simulink library "casper_library_pfbs"  (Simulink 7.2)
settings: Solver=ode45  SolverMode=SingleTasking  StartTime=0.0  StopTime=10.0  RelTol=1e-3
undefined symbols (not defined in the file or in its folder): pfb_coeff_gen_calc
libraries: xbsIndex_r4 x138, casper_library_pfbs x18, casper_library_delays x9, casper_library_misc x7, casper_library_flow_control x2
(part 3 of 3)

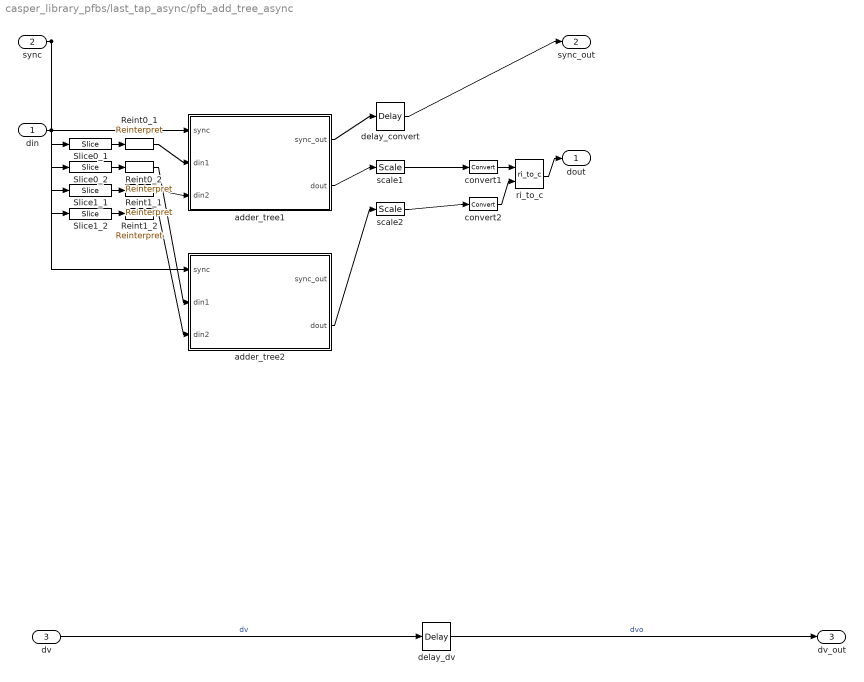
== system casper_library_pfbs/last_tap_async/pfb_add_tree_async ==
  din : Inport
  sync : Inport  Port=2
  dv : Inport  Port=3
  Reint0_1 : xbsIndex_r4/Reinterpret  force_arith_type=on  arith_type="Signed  (2's comp)"  force_bin_pt=on  bin_pt=coeff_bits + data_in_bits - 2  block_type=reinterpret
      settings: infoedit="Changes signal type without altering the binary representation.   You can changed the signal between signed and unsigned, and relocate the binary point.<br><br>Hardware notes: In hardware this block costs nothing.<br><br>Example:  Suppose the input is 6 bits wide, signed, with 2 fractional bits, and the output is forced to unsigned with 0 fractional bits.  Then an input of -2.0 (1110.00 in binary 2's complement) becomes an output of 56 (111000 in binary)."
  Reint0_2 : xbsIndex_r4/Reinterpret  force_arith_type=on  arith_type="Signed  (2's comp)"  force_bin_pt=on  bin_pt=coeff_bits + data_in_bits - 2  block_type=reinterpret
      settings: infoedit="Changes signal type without altering the binary representation.   You can changed the signal between signed and unsigned, and relocate the binary point.<br><br>Hardware notes: In hardware this block costs nothing.<br><br>Example:  Suppose the input is 6 bits wide, signed, with 2 fractional bits, and the output is forced to unsigned with 0 fractional bits.  Then an input of -2.0 (1110.00 in binary 2's complement) becomes an output of 56 (111000 in binary)."
  Reint1_1 : xbsIndex_r4/Reinterpret  force_arith_type=on  arith_type="Signed  (2's comp)"  force_bin_pt=on  bin_pt=coeff_bits + data_in_bits - 2  block_type=reinterpret
      settings: infoedit="Changes signal type without altering the binary representation.   You can changed the signal between signed and unsigned, and relocate the binary point.<br><br>Hardware notes: In hardware this block costs nothing.<br><br>Example:  Suppose the input is 6 bits wide, signed, with 2 fractional bits, and the output is forced to unsigned with 0 fractional bits.  Then an input of -2.0 (1110.00 in binary 2's complement) becomes an output of 56 (111000 in binary)."
  Reint1_2 : xbsIndex_r4/Reinterpret  force_arith_type=on  arith_type="Signed  (2's comp)"  force_bin_pt=on  bin_pt=coeff_bits + data_in_bits - 2  block_type=reinterpret
      settings: infoedit="Changes signal type without altering the binary representation.   You can changed the signal between signed and unsigned, and relocate the binary point.<br><br>Hardware notes: In hardware this block costs nothing.<br><br>Example:  Suppose the input is 6 bits wide, signed, with 2 fractional bits, and the output is forced to unsigned with 0 fractional bits.  Then an input of -2.0 (1110.00 in binary 2's complement) becomes an output of 56 (111000 in binary)."
  Slice0_1 : xbsIndex_r4/Slice  nbits=coeff_bits + data_in_bits  boolean_output=off  mode=Upper Bit Location + Width  bit1=0  base1=MSB of Input  bit0=0  base0=MSB of Input  dbl_ovrd=off  block_type=slice
  Slice0_2 : xbsIndex_r4/Slice  nbits=coeff_bits + data_in_bits  boolean_output=off  mode=Upper Bit Location + Width  bit1=-16  base1=MSB of Input  bit0=0  base0=MSB of Input  dbl_ovrd=off  block_type=slice
  Slice1_1 : xbsIndex_r4/Slice  nbits=coeff_bits + data_in_bits  boolean_output=off  mode=Upper Bit Location + Width  bit1=-32  base1=MSB of Input  bit0=0  base0=MSB of Input  dbl_ovrd=off  block_type=slice
  Slice1_2 : xbsIndex_r4/Slice  nbits=coeff_bits + data_in_bits  boolean_output=off  mode=Upper Bit Location + Width  bit1=-48  base1=MSB of Input  bit0=0  base0=MSB of Input  dbl_ovrd=off  block_type=slice
  adder_tree1 : Subsystem  AncestorBlock=casper_library_misc/adder_tree  mask(adder_tree){n_inputs=2, latency=add_latency, adder_imp=Fabric, first_stage_hdl=off}
      mask prompts: n_inputs "Number of Inputs"; latency "Add Latency"; adder_imp "Adder implementation"; first_stage_hdl "Use behavioural HDL for first stage of adders"
      mask help:
      | Sums all inputs using a tree of adds and delays.
      |
      | Number of inputs: The number of inputs to the block to be summed
      | Add latency: The number of clock cycles to perform one addition (affects timing)..
      | Adder implementation: choice of fabric or DSP48E core, or behavioral HDL
      | Use behavioural HDL for first stage of adders: Causes the first stage of adders to be absorbed into DSP blocks if multipliers precede them (Virtex 5). Overrides Adder implementation
      mask init:
      | adder_tree_init(gcb, ...
      |     'n_inputs', n_inputs, ...
      |     'latency', latency, ...
      |     'adder_imp', adder_imp, ...
      |     'first_stage_hdl', first_stage_hdl);
      settings: AttributesFormatString=latency 1
      mask Help: eval('xlWeb(''http://casper.berkeley.edu/wiki/Adder_tree'')')
      mask StyleString: edit,edit,popup(Behavioral|Fabric|DSP48),checkbox
  adder_tree2 : Subsystem  AncestorBlock=casper_library_misc/adder_tree  mask(adder_tree){n_inputs=2, latency=add_latency, adder_imp=Fabric, first_stage_hdl=off}
      mask prompts: n_inputs "Number of Inputs"; latency "Add Latency"; adder_imp "Adder implementation"; first_stage_hdl "Use behavioural HDL for first stage of adders"
      mask help:
      | Sums all inputs using a tree of adds and delays.
      |
      | Number of inputs: The number of inputs to the block to be summed
      | Add latency: The number of clock cycles to perform one addition (affects timing)..
      | Adder implementation: choice of fabric or DSP48E core, or behavioral HDL
      | Use behavioural HDL for first stage of adders: Causes the first stage of adders to be absorbed into DSP blocks if multipliers precede them (Virtex 5). Overrides Adder implementation
      mask init:
      | adder_tree_init(gcb, ...
      |     'n_inputs', n_inputs, ...
      |     'latency', latency, ...
      |     'adder_imp', adder_imp, ...
      |     'first_stage_hdl', first_stage_hdl);
      settings: AttributesFormatString=latency 1
      mask Help: eval('xlWeb(''http://casper.berkeley.edu/wiki/Adder_tree'')')
      mask StyleString: edit,edit,popup(Behavioral|Fabric|DSP48),checkbox
  convert1 : xbsIndex_r4/Convert  gui_display_data_type=Fixed-point  arith_type="Signed  (2's comp)"  n_bits=data_out_bits  bin_pt=data_out_bits-1  float_type=Single  exp_bits=8  fraction_bits=24  quantization=Truncate  overflow=Saturate  en=off  latency=add_latency  dbl_ovrd=off  pipeline=on  block_type=convert
      settings: block_version=11.4
  convert2 : xbsIndex_r4/Convert  gui_display_data_type=Fixed-point  arith_type="Signed  (2's comp)"  n_bits=data_out_bits  bin_pt=data_out_bits-1  float_type=Single  exp_bits=8  fraction_bits=24  quantization=Truncate  overflow=Saturate  en=off  latency=add_latency  dbl_ovrd=off  pipeline=on  block_type=convert
      settings: block_version=11.4
  delay_convert : xbsIndex_r4/Delay  rst=off  infoeditControl=Selection of Reset will increase slice count due to use of real FFs and instead of SRLs  en=off  latency=add_latency  dbl_ovrd=off  reg_retiming=off  block_type=delay
      settings: block_version=11.4
  delay_dv : xbsIndex_r4/Delay  rst=off  infoeditControl=Selection of Reset will increase slice count due to use of real FFs and instead of SRLs  en=off  latency=2  dbl_ovrd=off  reg_retiming=off  block_type=delay
      settings: block_version=11.4
  ri_to_c : casper_library_misc/ri_to_c
  scale1 : xbsIndex_r4/Scale  scale_factor=-2  dbl_ovrd=off  block_type=scale
  scale2 : xbsIndex_r4/Scale  scale_factor=-2  dbl_ovrd=off  block_type=scale
  dout : Outport
  sync_out : Outport  Port=2
  dv_out : Outport  Port=3
  wires:
  dv/1 -> delay_dv/1  "dv"
  delay_dv/1 -> dv_out/1  "dvo"
  adder_tree1/2(dout) -> scale1/1
  scale1/1 -> convert1/1
  adder_tree2/2(dout) -> scale2/1
  scale2/1 -> convert2/1
  convert1/1 -> ri_to_c/1
  convert2/1 -> ri_to_c/2
  ri_to_c/1 -> dout/1
  sync/1 -> adder_tree1/1(sync), adder_tree2/1(sync)
  adder_tree1/1(sync_out) -> delay_convert/1
  delay_convert/1 -> sync_out/1
  din/1 -> Slice0_1/1, Slice0_2/1, Slice1_1/1, Slice1_2/1
  Slice0_1/1 -> Reint0_1/1
  Reint0_1/1 -> adder_tree1/2(din1)
  Slice0_2/1 -> Reint0_2/1
  Reint0_2/1 -> adder_tree2/2(din1)
  Slice1_1/1 -> Reint1_1/1
  Reint1_1/1 -> adder_tree1/3(din2)
  Slice1_2/1 -> Reint1_2/1
  Reint1_2/1 -> adder_tree2/3(din2)

== system casper_library_pfbs/last_tap_async/ri_to_c ==
  re : Inport
  im : Inport  Port=2
  Concat : xbsIndex_r4/Concat  num_inputs=2  dbl_ovrd=off  block_type=concat
      settings: block_version=9.1.01
  Reinterpret : xbsIndex_r4/Reinterpret  force_arith_type=on  arith_type=Unsigned  force_bin_pt=on  bin_pt=0  block_type=reinterpret
      settings: infoedit="Changes signal type without altering the binary representation.   You can changed the signal between signed and unsigned, and relocate the binary point.<P><P>Hardware notes: In hardware this block costs nothing.<P><P>Example:  Suppose the input is 6 bits wide, signed, with 2 fractional bits, and the output is forced to unsigned with 0 fractional bits.  Then an input of -2.0 (1110.00 in binary 2's complement) becomes an output of 56 (111000 in binary)."  block_version=9.1.01
  Reinterpret1 : xbsIndex_r4/Reinterpret  force_arith_type=on  arith_type=Unsigned  force_bin_pt=on  bin_pt=0  block_type=reinterpret
      settings: infoedit="Changes signal type without altering the binary representation.   You can changed the signal between signed and unsigned, and relocate the binary point.<P><P>Hardware notes: In hardware this block costs nothing.<P><P>Example:  Suppose the input is 6 bits wide, signed, with 2 fractional bits, and the output is forced to unsigned with 0 fractional bits.  Then an input of -2.0 (1110.00 in binary 2's complement) becomes an output of 56 (111000 in binary)."  block_version=9.1.01
  c : Outport
  wires:
  im/1 -> Reinterpret1/1
  Concat/1 -> c/1
  re/1 -> Reinterpret/1
  Reinterpret1/1 -> Concat/2
  Reinterpret/1 -> Concat/1

== system casper_library_pfbs/pfb_fir_async/sync_generate ==
  sync : Inport
  dv : Inport  Port=2
  Constant : xbsIndex_r4/Constant  const=1  gui_display_data_type=Fixed-point  arith_type=Boolean  n_bits=16  bin_pt=14  preci_type=Single  exp_width=8  frac_width=24  explicit_period=on  period=1  equ=P=C  opselect=C  inp2=PCIN>>17  opr=+  inp1=P  carry=CIN  dbl_ovrd=off  block_type=constant
      settings: block_version=11.4
  Constant1 : xbsIndex_r4/Constant  const=(2^(pfb_bits - simul_bits) * (total_taps-1))+1  gui_display_data_type=Fixed-point  arith_type=Unsigned  n_bits=32  bin_pt=0  preci_type=Single  exp_width=8  frac_width=24  explicit_period=off  period=1  equ=P=C  opselect=C  inp2=PCIN>>17  opr=+  inp1=P  carry=CIN  dbl_ovrd=off  block_type=constant
      settings: block_version=11.4
  Counter : xbsIndex_r4/Counter  cnt_type=Free Running  cnt_to=Inf  operation=Up  start_count=0  cnt_by_val=1  arith_type=Unsigned  n_bits=32  bin_pt=0  load_pin=off  rst=on  en=on  explicit_period=on  period=1  dbl_ovrd=off  use_behavioral_HDL=off  implementation=Fabric  block_type=counter
      settings: block_version=11.4
  Logical : xbsIndex_r4/Logical  logical_function=AND  inputs=2  en=off  latency=0  precision=Full  arith_type=Unsigned  n_bits=16  bin_pt=0  align_bp=on  dbl_ovrd=off  block_type=logical
      settings: block_version=11.4
  Register : xbsIndex_r4/Register  init=0  rst=on  en=on  dbl_ovrd=off  block_type=register
      settings: block_version=11.4
  Relational : xbsIndex_r4/Relational  mode=a=b  en=off  latency=1  dbl_ovrd=off  block_type=relational
  sync_delay : xbsIndex_r4/Delay  rst=off  infoeditControl=Selection of Reset will increase slice count due to use of real FFs and instead of SRLs  en=off  latency=(bram_latency * (total_taps-1)) - 3  dbl_ovrd=off  reg_retiming=off  block_type=delay
      settings: block_version=11.4
  sync_out : Outport
  wires:
  sync_delay/1 -> sync_out/1
  dv/1 -> Logical/1
  sync/1 -> Register/3
  Relational/1 -> sync_delay/1, Counter/1, Register/2  "sync_out"
  Constant1/1 -> Relational/2
  Counter/1 -> Relational/1
  Logical/1 -> Counter/2
  Register/1 -> Logical/2
  Constant/1 -> Register/1

== system casper_library_pfbs/tap/ri_to_c ==
  re : Inport
  im : Inport  Port=2
  Concat : xbsIndex_r4/Concat  num_inputs=2  dbl_ovrd=off  block_type=concat
      settings: block_version=9.1.01
  Reinterpret : xbsIndex_r4/Reinterpret  force_arith_type=on  arith_type=Unsigned  force_bin_pt=on  bin_pt=0  block_type=reinterpret
      settings: infoedit="Changes signal type without altering the binary representation.   You can changed the signal between signed and unsigned, and relocate the binary point.<P><P>Hardware notes: In hardware this block costs nothing.<P><P>Example:  Suppose the input is 6 bits wide, signed, with 2 fractional bits, and the output is forced to unsigned with 0 fractional bits.  Then an input of -2.0 (1110.00 in binary 2's complement) becomes an output of 56 (111000 in binary)."  block_version=9.1.01
  Reinterpret1 : xbsIndex_r4/Reinterpret  force_arith_type=on  arith_type=Unsigned  force_bin_pt=on  bin_pt=0  block_type=reinterpret
      settings: infoedit="Changes signal type without altering the binary representation.   You can changed the signal between signed and unsigned, and relocate the binary point.<P><P>Hardware notes: In hardware this block costs nothing.<P><P>Example:  Suppose the input is 6 bits wide, signed, with 2 fractional bits, and the output is forced to unsigned with 0 fractional bits.  Then an input of -2.0 (1110.00 in binary 2's complement) becomes an output of 56 (111000 in binary)."  block_version=9.1.01
  c : Outport
  wires:
  im/1 -> Reinterpret1/1
  Concat/1 -> c/1
  re/1 -> Reinterpret/1
  Reinterpret1/1 -> Concat/2
  Reinterpret/1 -> Concat/1

== system casper_library_pfbs/tap_async/ri_to_c ==
  re : Inport
  im : Inport  Port=2
  Concat : xbsIndex_r4/Concat  num_inputs=2  dbl_ovrd=off  block_type=concat
      settings: block_version=9.1.01
  Reinterpret : xbsIndex_r4/Reinterpret  force_arith_type=on  arith_type=Unsigned  force_bin_pt=on  bin_pt=0  block_type=reinterpret
      settings: infoedit="Changes signal type without altering the binary representation.   You can changed the signal between signed and unsigned, and relocate the binary point.<P><P>Hardware notes: In hardware this block costs nothing.<P><P>Example:  Suppose the input is 6 bits wide, signed, with 2 fractional bits, and the output is forced to unsigned with 0 fractional bits.  Then an input of -2.0 (1110.00 in binary 2's complement) becomes an output of 56 (111000 in binary)."  block_version=9.1.01
  Reinterpret1 : xbsIndex_r4/Reinterpret  force_arith_type=on  arith_type=Unsigned  force_bin_pt=on  bin_pt=0  block_type=reinterpret
      settings: infoedit="Changes signal type without altering the binary representation.   You can changed the signal between signed and unsigned, and relocate the binary point.<P><P>Hardware notes: In hardware this block costs nothing.<P><P>Example:  Suppose the input is 6 bits wide, signed, with 2 fractional bits, and the output is forced to unsigned with 0 fractional bits.  Then an input of -2.0 (1110.00 in binary 2's complement) becomes an output of 56 (111000 in binary)."  block_version=9.1.01
  c : Outport
  wires:
  Reinterpret/1 -> Concat/1
  Reinterpret1/1 -> Concat/2
  re/1 -> Reinterpret/1
  Concat/1 -> c/1
  im/1 -> Reinterpret1/1

== system casper_library_pfbs/last_tap/pfb_add_tree/adder_tree1 ==
  sync : Inport
  din1 : Inport  Port=2
  din2 : Inport  Port=3
  din3 : Inport  Port=4
  din4 : Inport  Port=5
  addr1 : xbsIndex_r4/AddSub  mode=Addition  use_carryin=off  use_carryout=off  en=off  latency=1  precision=Full  arith_type=Unsigned  n_bits=16  bin_pt=14  quantization=Truncate  overflow=Wrap  dbl_ovrd=off  use_behavioral_HDL=off  hw_selection=Fabric  pipelined=on  use_rpm=on  block_type=addsub
  addr2 : xbsIndex_r4/AddSub  mode=Addition  use_carryin=off  use_carryout=off  en=off  latency=1  precision=Full  arith_type=Unsigned  n_bits=16  bin_pt=14  quantization=Truncate  overflow=Wrap  dbl_ovrd=off  use_behavioral_HDL=off  hw_selection=Fabric  pipelined=on  use_rpm=on  block_type=addsub
  addr3 : xbsIndex_r4/AddSub  mode=Addition  use_carryin=off  use_carryout=off  en=off  latency=1  precision=Full  arith_type=Unsigned  n_bits=16  bin_pt=14  quantization=Truncate  overflow=Wrap  dbl_ovrd=off  use_behavioral_HDL=off  hw_selection=Fabric  pipelined=on  use_rpm=on  block_type=addsub
  sync_delay : xbsIndex_r4/Delay  rst=off  infoeditControl=Selection of Reset will increase slice count due to use of real FFs and instead of SRLs  en=off  latency=2  dbl_ovrd=off  reg_retiming=on  block_type=delay
      settings: block_version=11.4
  sync_out : Outport
  dout : Outport  Port=2
  wires:
  sync/1 -> sync_delay/1
  sync_delay/1 -> sync_out/1
  din1/1 -> addr1/1
  din2/1 -> addr1/2
  din3/1 -> addr2/1
  din4/1 -> addr2/2
  addr1/1 -> addr3/1
  addr2/1 -> addr3/2
  addr3/1 -> dout/1

== system casper_library_pfbs/last_tap/pfb_add_tree/adder_tree2 ==
  sync : Inport
  din1 : Inport  Port=2
  din2 : Inport  Port=3
  din3 : Inport  Port=4
  din4 : Inport  Port=5
  addr1 : xbsIndex_r4/AddSub  mode=Addition  use_carryin=off  use_carryout=off  en=off  latency=1  precision=Full  arith_type=Unsigned  n_bits=16  bin_pt=14  quantization=Truncate  overflow=Wrap  dbl_ovrd=off  use_behavioral_HDL=off  hw_selection=Fabric  pipelined=on  use_rpm=on  block_type=addsub
  addr2 : xbsIndex_r4/AddSub  mode=Addition  use_carryin=off  use_carryout=off  en=off  latency=1  precision=Full  arith_type=Unsigned  n_bits=16  bin_pt=14  quantization=Truncate  overflow=Wrap  dbl_ovrd=off  use_behavioral_HDL=off  hw_selection=Fabric  pipelined=on  use_rpm=on  block_type=addsub
  addr3 : xbsIndex_r4/AddSub  mode=Addition  use_carryin=off  use_carryout=off  en=off  latency=1  precision=Full  arith_type=Unsigned  n_bits=16  bin_pt=14  quantization=Truncate  overflow=Wrap  dbl_ovrd=off  use_behavioral_HDL=off  hw_selection=Fabric  pipelined=on  use_rpm=on  block_type=addsub
  sync_delay : xbsIndex_r4/Delay  rst=off  infoeditControl=Selection of Reset will increase slice count due to use of real FFs and instead of SRLs  en=off  latency=2  dbl_ovrd=off  reg_retiming=on  block_type=delay
      settings: block_version=11.4
  sync_out : Outport
  dout : Outport  Port=2
  wires:
  sync/1 -> sync_delay/1
  sync_delay/1 -> sync_out/1
  din1/1 -> addr1/1
  din2/1 -> addr1/2
  din3/1 -> addr2/1
  din4/1 -> addr2/2
  addr1/1 -> addr3/1
  addr2/1 -> addr3/2
  addr3/1 -> dout/1

== system casper_library_pfbs/last_tap_async/pfb_add_tree_async/adder_tree1 ==
  sync : Inport
  din1 : Inport  Port=2
  din2 : Inport  Port=3
  addr1 : xbsIndex_r4/AddSub  mode=Addition  use_carryin=off  use_carryout=off  en=off  latency=1  precision=Full  arith_type=Unsigned  n_bits=16  bin_pt=14  quantization=Truncate  overflow=Wrap  dbl_ovrd=off  use_behavioral_HDL=off  hw_selection=Fabric  pipelined=on  use_rpm=on  block_type=addsub
  sync_delay : xbsIndex_r4/Delay  rst=off  infoeditControl=Selection of Reset will increase slice count due to use of real FFs and instead of SRLs  en=off  latency=1  dbl_ovrd=off  reg_retiming=on  block_type=delay
      settings: block_version=11.4
  sync_out : Outport
  dout : Outport  Port=2
  wires:
  sync/1 -> sync_delay/1
  sync_delay/1 -> sync_out/1
  din1/1 -> addr1/1
  din2/1 -> addr1/2
  addr1/1 -> dout/1

== system casper_library_pfbs/last_tap_async/pfb_add_tree_async/adder_tree2 ==
  sync : Inport
  din1 : Inport  Port=2
  din2 : Inport  Port=3
  addr1 : xbsIndex_r4/AddSub  mode=Addition  use_carryin=off  use_carryout=off  en=off  latency=1  precision=Full  arith_type=Unsigned  n_bits=16  bin_pt=14  quantization=Truncate  overflow=Wrap  dbl_ovrd=off  use_behavioral_HDL=off  hw_selection=Fabric  pipelined=on  use_rpm=on  block_type=addsub
  sync_delay : xbsIndex_r4/Delay  rst=off  infoeditControl=Selection of Reset will increase slice count due to use of real FFs and instead of SRLs  en=off  latency=1  dbl_ovrd=off  reg_retiming=on  block_type=delay
      settings: block_version=11.4
  sync_out : Outport
  dout : Outport  Port=2
  wires:
  sync/1 -> sync_delay/1
  sync_delay/1 -> sync_out/1
  din1/1 -> addr1/1
  din2/1 -> addr1/2
  addr1/1 -> dout/1
